simulink library "casper_library_delays"  (Simulink 7.2)
settings: Solver=ode45  SolverMode=SingleTasking  StartTime=0.0  StopTime=10.0  RelTol=1e-3
libraries: xbsIndex_r4 x378, casper_library_misc x18, casper_library_delays x16, xbsReplacements_r4 x5, casper_library_multipliers x4, casper_library_downconverter x2
(part 3 of 5)

== system casper_library_delays/finedelay_fstop_prog_cordic/CORDIC_SINCOS2 ==
  note: The CORDIC algorithm is implemented in 3 steps.
      |
      | Step 1: Coarse Angle Rotation.  The algorithm converges only for angles between -pi/2 and pi/2. If  z > pi/2, the input angle is reflected
      |  to the 1st quadrant by subtracting pi/2 from the input angle. When z < -pi/2, the input angle is reflected back to the 3rd quadrant by adding
      | pi/2 to the input angle .
      |
      | Step 2: Fine Angle Rotation.  By setting x equal to 1/1.646760 and y equal to 0, the rotational mode CORDIC processor yields cosine and sine
      | of the input angle Z.
      |
      | Step 3: Angle Correction. If there was a reflection applied in Step 1, this step applies the appropriate correction .
  z : Inport
  CORDIC Fine Angle PE : Subsystem  mask(CORDIC parallel PE){}
      mask init:
      | [bg,fg] = xlcmap('XBlock',0);
      | iPos = get_param(gcb,'Position');
      | iWidth=iPos(3)-iPos(1); iHeight=iPos(4)-iPos(2);
      | iCx=iWidth/2;
      | iCy=iHeight/2;
      | [logoX, logoY] = xlogo(iPos);
      mask Display:
      | patch([0 iWidth iWidth 0],[0 0 iHeight iHeight] , bg);
      | patch(logoX,logoY , fg);
      | port_label('input',1,'x');
      | port_label('input',2,'y');
      | port_label('input',3,'z');
      | port_label('output',1,'X');
      | port_label('output',2,'Y');
      | plot([0 0 iWidth iWidth 0], [0 iHeight iHeight 0 0]);
  Constant : xbsIndex_r4/Constant  const=1/1.646760  gui_display_data_type=Fixed-point  arith_type=Signed (2's comp)  n_bits=pe_nbits  bin_pt=pe_binpt  preci_type=Single  exp_width=8  frac_width=24  explicit_period=off  period=1  equ=P=C  opselect=C  inp2=PCIN>>17  opr=+  inp1=P  carry=CIN  dbl_ovrd=off  block_type=constant
      settings: block_version=VER_STRING_GOES_HERE
  Constant1 : xbsIndex_r4/Constant  const=0  gui_display_data_type=Fixed-point  arith_type=Signed (2's comp)  n_bits=pe_nbits  bin_pt=pe_binpt  preci_type=Single  exp_width=8  frac_width=24  explicit_period=off  period=1  equ=P=C  opselect=C  inp2=PCIN>>17  opr=+  inp1=P  carry=CIN  dbl_ovrd=off  block_type=constant
      settings: block_version=VER_STRING_GOES_HERE
  Delay1 : xbsIndex_r4/Delay  rst=off  infoeditControl=Selection of Reset will increase slice count due to use of real FFs and instead of SRLs  en=off  latency=sum(pipeline)+2  dbl_ovrd=off  reg_retiming=on  block_type=delay
      settings: infoedit="Delay line having  configurable length.<P><P>Hardware notes: A delay line is a chain, each link of which is an SRL16 followed by a flip-flop. If register retiming is enabled, the delay line is a chain of flip-flops."  xl_area=[1 1 0 1 0 0 0]  block_version=VER_STRING_GOES_HERE
  Delay4 : xbsIndex_r4/Delay  rst=off  infoeditControl=Selection of Reset will increase slice count due to use of real FFs and instead of SRLs  en=off  latency=sum(pipeline)+1  dbl_ovrd=off  reg_retiming=on  block_type=delay
      settings: infoedit="Delay line having  configurable length.<P><P>Hardware notes: A delay line is a chain, each link of which is an SRL16 followed by a flip-flop. If register retiming is enabled, the delay line is a chain of flip-flops."  xl_area=[1 1 0 1 0 0 0]  block_version=VER_STRING_GOES_HERE
  Quadrant Correct : Subsystem
      mask init:
      | [bg,fg] = xlcmap('XBlock',0);
      | iPos = get_param(gcb,'Position');
      | iWidth=iPos(3)-iPos(1); iHeight=iPos(4)-iPos(2);
      | iCx=iWidth/2;
      | iCy=iHeight/2;
      | [logoX, logoY] = xlogo(iPos);
      mask Display:
      | patch([0 iWidth iWidth 0],[0 0 iHeight iHeight] , bg);
      | patch(logoX,logoY , fg);
      | port_label('input',1,'x');
      | port_label('input',2,'y');
      | port_label('input',3,'angle_map');
      | port_label('input',4,'sgn(z)');
      | port_label('output',1,'cos');
      | port_label('output',2,'sin');
      | plot([0 0 iWidth iWidth 0], [0 iHeight iHeight 0 0]);
  Quadrant Map : Subsystem
      mask init:
      | [bg,fg] = xlcmap('XBlock',0);
      | iPos = get_param(gcb,'Position');
      | iWidth=iPos(3)-iPos(1); iHeight=iPos(4)-iPos(2);
      | iCx=iWidth/2;
      | iCy=iHeight/2;
      | [logoX, logoY] = xlogo(iPos);
      mask Display:
      | patch([0 iWidth iWidth 0],[0 0 iHeight iHeight] , bg);
      | patch(logoX,logoY , fg);
      | port_label('input',1,'z');
      | port_label('output',1,'z');
      | port_label('output',2,'angle_map');
      | port_label('output',3,'sgn(z)');
      | plot([0 0 iWidth iWidth 0], [0 iHeight iHeight 0 0]);
  cos : Outport
  sin : Outport  Port=2
  wires:
  CORDIC Fine Angle PE/1(X) -> Quadrant Correct/1(cos)
  CORDIC Fine Angle PE/2(Y) -> Quadrant Correct/2(sin)
  Delay1/1 -> Quadrant Correct/4(sgn(z))
  Delay4/1 -> Quadrant Correct/3(angle_map)
  z/1 -> Quadrant Map/1(z)
  Quadrant Map/2(angle_map) -> Delay4/1
  Quadrant Map/3(sgn_z) -> Delay1/1
  Quadrant Map/1(Z) -> CORDIC Fine Angle PE/3(z)
  Constant/1 -> CORDIC Fine Angle PE/1(x)
  Constant1/1 -> CORDIC Fine Angle PE/2(y)
  Quadrant Correct/2(sine) -> sin/1
  Quadrant Correct/1(cosine) -> cos/1

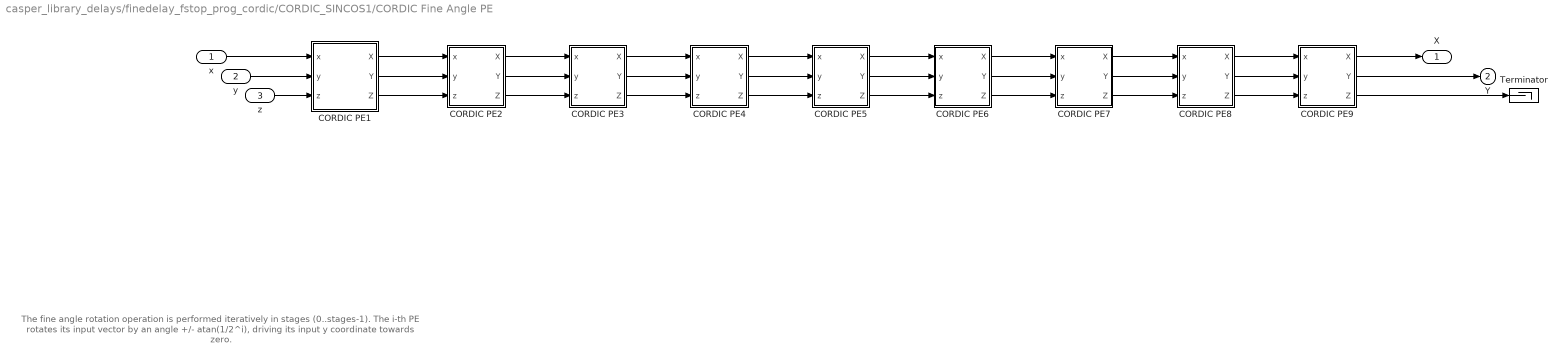
== system casper_library_delays/finedelay_fstop_prog_cordic/CORDIC_SINCOS1/CORDIC Fine Angle PE ==
  note: The fine angle rotation operation is performed iteratively in stages (0..stages-1).
      | The i-th PE rotates its input vector by an angle +/- atan(1/2^i), driving its input y coordinate towards zero.
  x : Inport
  y : Inport  Port=2
  z : Inport  Port=3
  CORDIC PE1 : Subsystem  mask(CORDIC iteration PE){ii=0, pe_nbits=pe_nbits, pe_binpt=pe_binpt, epsilon_k_fcn=atan, epsilon_k=, pipeline=pipeline(1,1)}
      mask prompts: ii "Iteration Index ii"; pe_nbits "Number of X,Y,Z Bits"; pe_binpt "X,Y,Z Binary Point Position"; epsilon_k_fcn "Epsilon_k Function"; pipeline "Pipeline Latency"
      mask init:
      | [bg,fg] = xlcmap('XBlock',0);
      | iPos = get_param(gcb,'Position');
      | iWidth=iPos(3)-iPos(1); iHeight=iPos(4)-iPos(2);
      | iCx=iWidth/2;
      | iCy=iHeight/2;
      | [logoX, logoY] = xlogo(iPos);
      | 
      | set_param(gcb, 'LinkStatus', 'none');
      | switch epsilon_k_fcn
      |   case 1
      |     epsilon_k = atan(1/2^ii);
      |   case 2
      |     epsilon_k = atanh(1/2^ii);
      | end
      mask StyleString: edit,edit,edit,popup(atan|atanh),edit,edit
      mask Display:
      | patch([0 iWidth iWidth 0],[0 0 iHeight iHeight] , bg);
      | patch(logoX,logoY , fg);
      | port_label('input',1,'x');
      | port_label('input',2,'y');
      | port_label('input',3,'z');
      | port_label('output',1,'X');
      | port_label('output',2,'Y');
      | port_label('output',3,'Z');
      | plot([0 0 iWidth iWidth 0], [0 iHeight iHeight 0 0]);
  CORDIC PE2 : Subsystem  mask(CORDIC iteration PE){ii=1, pe_nbits=pe_nbits, pe_binpt=pe_binpt, epsilon_k_fcn=atan, epsilon_k=, pipeline=pipeline(1,2)}
      mask prompts: ii "Iteration Index ii"; pe_nbits "Number of X,Y,Z Bits"; pe_binpt "X,Y,Z Binary Point Position"; epsilon_k_fcn "Epsilon_k Function"; pipeline "Pipeline Latency"
      mask init: same as casper_library_delays/finedelay_fstop_prog_cordic/CORDIC_SINCOS1/CORDIC Fine Angle PE/CORDIC PE1
      mask StyleString: edit,edit,edit,popup(atan|atanh),edit,edit
      mask Display:
      | patch([0 iWidth iWidth 0],[0 0 iHeight iHeight] , bg);
      | patch(logoX,logoY , fg);
      | port_label('input',1,'x');
      | port_label('input',2,'y');
      | port_label('input',3,'z');
      | port_label('output',1,'X');
      | port_label('output',2,'Y');
      | port_label('output',3,'Z');
      | plot([0 0 iWidth iWidth 0], [0 iHeight iHeight 0 0]);
  CORDIC PE3 : Subsystem  mask(CORDIC iteration PE){ii=2, pe_nbits=pe_nbits, pe_binpt=pe_binpt, epsilon_k_fcn=atan, epsilon_k=, pipeline=pipeline(1,3)}
      mask prompts: ii "Iteration Index ii"; pe_nbits "Number of X,Y,Z Bits"; pe_binpt "X,Y,Z Binary Point Position"; epsilon_k_fcn "Epsilon_k Function"; pipeline "Pipeline Latency"
      mask init: same as casper_library_delays/finedelay_fstop_prog_cordic/CORDIC_SINCOS1/CORDIC Fine Angle PE/CORDIC PE1
      mask StyleString: edit,edit,edit,popup(atan|atanh),edit,edit
      mask Display:
      | patch([0 iWidth iWidth 0],[0 0 iHeight iHeight] , bg);
      | patch(logoX,logoY , fg);
      | port_label('input',1,'x');
      | port_label('input',2,'y');
      | port_label('input',3,'z');
      | port_label('output',1,'X');
      | port_label('output',2,'Y');
      | port_label('output',3,'Z');
      | plot([0 0 iWidth iWidth 0], [0 iHeight iHeight 0 0]);
  CORDIC PE4 : Subsystem  mask(CORDIC iteration PE){ii=3, pe_nbits=pe_nbits, pe_binpt=pe_binpt, epsilon_k_fcn=atan, epsilon_k=, pipeline=pipeline(1,4)}
      mask prompts: ii "Iteration Index ii"; pe_nbits "Number of X,Y,Z Bits"; pe_binpt "X,Y,Z Binary Point Position"; epsilon_k_fcn "Epsilon_k Function"; pipeline "Pipeline Latency"
      mask init: same as casper_library_delays/finedelay_fstop_prog_cordic/CORDIC_SINCOS1/CORDIC Fine Angle PE/CORDIC PE1
      mask StyleString: edit,edit,edit,popup(atan|atanh),edit,edit
      mask Display:
      | patch([0 iWidth iWidth 0],[0 0 iHeight iHeight] , bg);
      | patch(logoX,logoY , fg);
      | port_label('input',1,'x');
      | port_label('input',2,'y');
      | port_label('input',3,'z');
      | port_label('output',1,'X');
      | port_label('output',2,'Y');
      | port_label('output',3,'Z');
      | plot([0 0 iWidth iWidth 0], [0 iHeight iHeight 0 0]);
  CORDIC PE5 : Subsystem  mask(CORDIC iteration PE){ii=4, pe_nbits=pe_nbits, pe_binpt=pe_binpt, epsilon_k_fcn=atan, epsilon_k=, pipeline=pipeline(1,5)}
      mask prompts: ii "Iteration Index ii"; pe_nbits "Number of X,Y,Z Bits"; pe_binpt "X,Y,Z Binary Point Position"; epsilon_k_fcn "Epsilon_k Function"; pipeline "Pipeline Latency"
      mask init: same as casper_library_delays/finedelay_fstop_prog_cordic/CORDIC_SINCOS1/CORDIC Fine Angle PE/CORDIC PE1
      mask StyleString: edit,edit,edit,popup(atan|atanh),edit,edit
      mask Display:
      | patch([0 iWidth iWidth 0],[0 0 iHeight iHeight] , bg);
      | patch(logoX,logoY , fg);
      | port_label('input',1,'x');
      | port_label('input',2,'y');
      | port_label('input',3,'z');
      | port_label('output',1,'X');
      | port_label('output',2,'Y');
      | port_label('output',3,'Z');
      | plot([0 0 iWidth iWidth 0], [0 iHeight iHeight 0 0]);
  CORDIC PE6 : Subsystem  mask(CORDIC iteration PE){ii=5, pe_nbits=pe_nbits, pe_binpt=pe_binpt, epsilon_k_fcn=atan, epsilon_k=, pipeline=pipeline(1,6)}
      mask prompts: ii "Iteration Index ii"; pe_nbits "Number of X,Y,Z Bits"; pe_binpt "X,Y,Z Binary Point Position"; epsilon_k_fcn "Epsilon_k Function"; pipeline "Pipeline Latency"
      mask init: same as casper_library_delays/finedelay_fstop_prog_cordic/CORDIC_SINCOS1/CORDIC Fine Angle PE/CORDIC PE1
      mask StyleString: edit,edit,edit,popup(atan|atanh),edit,edit
      mask Display:
      | patch([0 iWidth iWidth 0],[0 0 iHeight iHeight] , bg);
      | patch(logoX,logoY , fg);
      | port_label('input',1,'x');
      | port_label('input',2,'y');
      | port_label('input',3,'z');
      | port_label('output',1,'X');
      | port_label('output',2,'Y');
      | port_label('output',3,'Z');
      | plot([0 0 iWidth iWidth 0], [0 iHeight iHeight 0 0]);
  CORDIC PE7 : Subsystem  mask(CORDIC iteration PE){ii=6, pe_nbits=pe_nbits, pe_binpt=pe_binpt, epsilon_k_fcn=atan, epsilon_k=, pipeline=pipeline(1,7)}
      mask prompts: ii "Iteration Index ii"; pe_nbits "Number of X,Y,Z Bits"; pe_binpt "X,Y,Z Binary Point Position"; epsilon_k_fcn "Epsilon_k Function"; pipeline "Pipeline Latency"
      mask init: same as casper_library_delays/finedelay_fstop_prog_cordic/CORDIC_SINCOS1/CORDIC Fine Angle PE/CORDIC PE1
      mask StyleString: edit,edit,edit,popup(atan|atanh),edit,edit
      mask Display:
      | patch([0 iWidth iWidth 0],[0 0 iHeight iHeight] , bg);
      | patch(logoX,logoY , fg);
      | port_label('input',1,'x');
      | port_label('input',2,'y');
      | port_label('input',3,'z');
      | port_label('output',1,'X');
      | port_label('output',2,'Y');
      | port_label('output',3,'Z');
      | plot([0 0 iWidth iWidth 0], [0 iHeight iHeight 0 0]);
  CORDIC PE8 : Subsystem  mask(CORDIC iteration PE){ii=7, pe_nbits=pe_nbits, pe_binpt=pe_binpt, epsilon_k_fcn=atan, epsilon_k=, pipeline=pipeline(1,8)}
      mask prompts: ii "Iteration Index ii"; pe_nbits "Number of X,Y,Z Bits"; pe_binpt "X,Y,Z Binary Point Position"; epsilon_k_fcn "Epsilon_k Function"; pipeline "Pipeline Latency"
      mask init: same as casper_library_delays/finedelay_fstop_prog_cordic/CORDIC_SINCOS1/CORDIC Fine Angle PE/CORDIC PE1
      mask StyleString: edit,edit,edit,popup(atan|atanh),edit,edit
      mask Display:
      | patch([0 iWidth iWidth 0],[0 0 iHeight iHeight] , bg);
      | patch(logoX,logoY , fg);
      | port_label('input',1,'x');
      | port_label('input',2,'y');
      | port_label('input',3,'z');
      | port_label('output',1,'X');
      | port_label('output',2,'Y');
      | port_label('output',3,'Z');
      | plot([0 0 iWidth iWidth 0], [0 iHeight iHeight 0 0]);
  CORDIC PE9 : Subsystem  mask(CORDIC iteration PE){ii=8, pe_nbits=pe_nbits, pe_binpt=pe_binpt, epsilon_k_fcn=atan, epsilon_k=, pipeline=pipeline(1,9)}
      mask prompts: ii "Iteration Index ii"; pe_nbits "Number of X,Y,Z Bits"; pe_binpt "X,Y,Z Binary Point Position"; epsilon_k_fcn "Epsilon_k Function"; pipeline "Pipeline Latency"
      mask init: same as casper_library_delays/finedelay_fstop_prog_cordic/CORDIC_SINCOS1/CORDIC Fine Angle PE/CORDIC PE1
      mask StyleString: edit,edit,edit,popup(atan|atanh),edit,edit
      mask Display:
      | patch([0 iWidth iWidth 0],[0 0 iHeight iHeight] , bg);
      | patch(logoX,logoY , fg);
      | port_label('input',1,'x');
      | port_label('input',2,'y');
      | port_label('input',3,'z');
      | port_label('output',1,'X');
      | port_label('output',2,'Y');
      | port_label('output',3,'Z');
      | plot([0 0 iWidth iWidth 0], [0 iHeight iHeight 0 0]);
  Terminator : Terminator
  X : Outport
  Y : Outport  Port=2
  wires:
  CORDIC PE1/1(X) -> CORDIC PE2/1(x)
  CORDIC PE1/2(Y) -> CORDIC PE2/2(y)
  CORDIC PE1/3(Z) -> CORDIC PE2/3(z)
  CORDIC PE2/1(X) -> CORDIC PE3/1(x)
  CORDIC PE2/2(Y) -> CORDIC PE3/2(y)
  CORDIC PE2/3(Z) -> CORDIC PE3/3(z)
  CORDIC PE3/1(X) -> CORDIC PE4/1(x)
  CORDIC PE3/2(Y) -> CORDIC PE4/2(y)
  CORDIC PE3/3(Z) -> CORDIC PE4/3(z)
  CORDIC PE4/1(X) -> CORDIC PE5/1(x)
  CORDIC PE4/2(Y) -> CORDIC PE5/2(y)
  CORDIC PE4/3(Z) -> CORDIC PE5/3(z)
  CORDIC PE5/1(X) -> CORDIC PE6/1(x)
  CORDIC PE5/2(Y) -> CORDIC PE6/2(y)
  CORDIC PE5/3(Z) -> CORDIC PE6/3(z)
  CORDIC PE6/1(X) -> CORDIC PE7/1(x)
  CORDIC PE6/2(Y) -> CORDIC PE7/2(y)
  CORDIC PE6/3(Z) -> CORDIC PE7/3(z)
  CORDIC PE7/1(X) -> CORDIC PE8/1(x)
  CORDIC PE7/2(Y) -> CORDIC PE8/2(y)
  CORDIC PE7/3(Z) -> CORDIC PE8/3(z)
  CORDIC PE8/1(X) -> CORDIC PE9/1(x)
  CORDIC PE8/2(Y) -> CORDIC PE9/2(y)
  CORDIC PE8/3(Z) -> CORDIC PE9/3(z)
  x/1 -> CORDIC PE1/1(x)
  y/1 -> CORDIC PE1/2(y)
  z/1 -> CORDIC PE1/3(z)
  CORDIC PE9/1(X) -> X/1
  CORDIC PE9/2(Y) -> Y/1
  CORDIC PE9/3(Z) -> Terminator/1

== system casper_library_delays/finedelay_fstop_prog_cordic/CORDIC_SINCOS1/Quadrant Correct ==
  note: Angle Correction:
      |
      | IF z > pi/2: using z = t + pi/2, then
      |    sin (z ) = sin(t).cos(pi/2) + cos(t).sin(pi/2) = cos(t)
      |    cos (z ) = cos(t).cos(pi/2) - sin(t).sin(pi/2) = -sin(t)
      |
      | IF z < pi/2: using z = t - pi/2, then
      |    sin (z ) = sin(t).cos(-pi/2) + cos(t).sin(-pi/2) = -cos(t)
      |    cos (z ) = cos(t).cos(-pi/2) - sin(t).sin(-pi/2) = sin(t)
  cos : Inport
  sin : Inport  Port=2
  angle_map : Inport  Port=3
  sgn(z) : Inport  Port=4
  Mux : xbsIndex_r4/Mux  inputs=2  en=off  latency=1  precision=User Defined  arith_type="Signed  (2's comp)"  n_bits=pe_nbits  bin_pt=pe_binpt  quantization=Truncate  overflow=Wrap  dbl_ovrd=off  block_type=mux
      settings: xl_area=[8 16 0 16 0 0 0]  block_version=VER_STRING_GOES_HERE
  Mux1 : xbsIndex_r4/Mux  inputs=2  en=off  latency=1  precision=User Defined  arith_type="Signed  (2's comp)"  n_bits=pe_nbits  bin_pt=pe_binpt  quantization=Truncate  overflow=Wrap  dbl_ovrd=off  block_type=mux
      settings: xl_area=[8 16 0 16 0 0 0]  block_version=VER_STRING_GOES_HERE
  Mux2 : xbsIndex_r4/Mux  inputs=2  en=off  latency=0  precision=User Defined  arith_type="Signed  (2's comp)"  n_bits=pe_nbits  bin_pt=pe_binpt  quantization=Truncate  overflow=Wrap  dbl_ovrd=off  block_type=mux
      settings: xl_area=[8 0 0 16 0 0 0]  block_version=VER_STRING_GOES_HERE
  Mux3 : xbsIndex_r4/Mux  inputs=2  en=off  latency=0  precision=User Defined  arith_type="Signed  (2's comp)"  n_bits=pe_nbits  bin_pt=pe_binpt  quantization=Truncate  overflow=Wrap  dbl_ovrd=off  block_type=mux
      settings: xl_area=[8 0 0 16 0 0 0]  block_version=VER_STRING_GOES_HERE
  Negate1 : xbsIndex_r4/Negate  precision=User Defined  arith_type="Signed  (2's comp)"  n_bits=pe_nbits  bin_pt=pe_binpt  quantization=Truncate  overflow=Wrap  en=off  latency=0  dbl_ovrd=off  block_type=negate
      settings: xl_area=[8 0 0 16 0 0 0]  block_version=VER_STRING_GOES_HERE
  Negate2 : xbsIndex_r4/Negate  precision=User Defined  arith_type="Signed  (2's comp)"  n_bits=pe_nbits  bin_pt=pe_binpt  quantization=Truncate  overflow=Wrap  en=off  latency=0  dbl_ovrd=off  block_type=negate
      settings: xl_area=[8 0 0 16 0 0 0]  block_version=VER_STRING_GOES_HERE
  cosine : Outport
  sine : Outport  Port=2
  wires:
  cos/1 -> Mux/2, Negate1/1, Mux2/2
  sin/1 -> Mux1/2, Negate2/1, Mux3/3
  Mux/1 -> cosine/1
  Mux1/1 -> sine/1
  angle_map/1 -> Mux/1, Mux1/1
  Mux3/1 -> Mux/3
  sgn(z)/1 -> Mux2/1, Mux3/1
  Mux2/1 -> Mux1/3
  Negate1/1 -> Mux2/3
  Negate2/1 -> Mux3/2

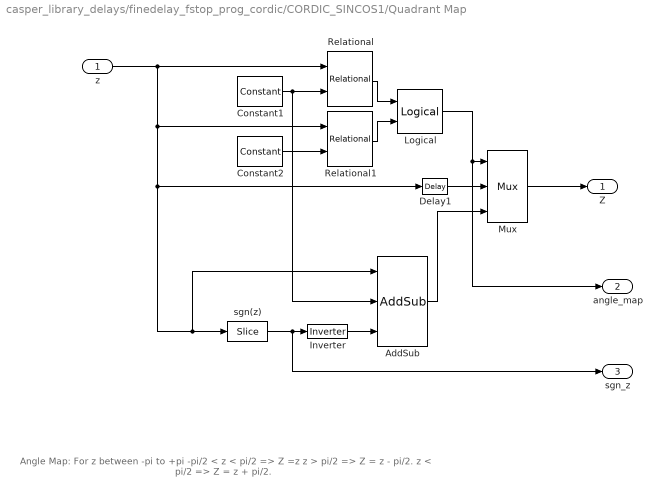
== system casper_library_delays/finedelay_fstop_prog_cordic/CORDIC_SINCOS1/Quadrant Map ==
  note: Angle Map: For z between -pi to +pi
      |
      |  -pi/2 < z  < pi/2  =>  Z =z
      |             z > pi/2   =>  Z = z - pi/2.
      |             z < pi/2   =>  Z = z + pi/2.
  z : Inport
  AddSub : xbsIndex_r4/AddSub  mode=Addition or Subtraction  use_carryin=off  use_carryout=off  en=off  latency=1  precision=User Defined  arith_type="Signed  (2's comp)"  n_bits=pe_nbits  bin_pt=pe_binpt  quantization=Truncate  overflow=Wrap  dbl_ovrd=off  use_behavioral_HDL=on  hw_selection=Fabric  pipelined=off  use_rpm=off  block_type=addsub
      settings: xl_area=[8 16 0 16 0 0 0]  block_version=VER_STRING_GOES_HERE
  Constant1 : xbsIndex_r4/Constant  const=pi/2  gui_display_data_type=Fixed-point  arith_type=Signed (2's comp)  n_bits=pe_nbits  bin_pt=pe_binpt  preci_type=Single  exp_width=8  frac_width=24  explicit_period=off  period=1  equ=P=C  opselect=C  inp2=PCIN>>17  opr=+  inp1=P  carry=CIN  dbl_ovrd=off  block_type=constant
      settings: block_version=VER_STRING_GOES_HERE
  Constant2 : xbsIndex_r4/Constant  const=-pi/2  gui_display_data_type=Fixed-point  arith_type=Signed (2's comp)  n_bits=pe_nbits  bin_pt=pe_binpt  preci_type=Single  exp_width=8  frac_width=24  explicit_period=off  period=1  equ=P=C  opselect=C  inp2=PCIN>>17  opr=+  inp1=P  carry=CIN  dbl_ovrd=off  block_type=constant
      settings: block_version=VER_STRING_GOES_HERE
  Delay1 : xbsIndex_r4/Delay  rst=off  infoeditControl=Selection of Reset will increase slice count due to use of real FFs and instead of SRLs  en=off  latency=1  dbl_ovrd=off  reg_retiming=on  block_type=delay
      settings: infoedit="Delay line having  configurable length.<P><P>Hardware notes: A delay line is a chain, each link of which is an SRL16 followed by a flip-flop. If register retiming is enabled, the delay line is a chain of flip-flops."  xl_area=[8 16 0 0 0 0 0]  block_version=VER_STRING_GOES_HERE
  Inverter : xbsIndex_r4/Inverter  en=off  latency=0  dbl_ovrd=off  block_type=inv
      settings: xl_area=[1 0 0 1 0 0 0]  block_version=VER_STRING_GOES_HERE
  Logical : xbsIndex_r4/Logical  logical_function=OR  inputs=2  en=off  latency=0  precision=Full  arith_type=Unsigned  n_bits=8  bin_pt=2  align_bp=on  dbl_ovrd=off  block_type=logical
      settings: xl_area=[1 0 0 1 0 0 0]  block_version=VER_STRING_GOES_HERE
  Mux : xbsIndex_r4/Mux  inputs=2  en=off  latency=1  precision=User Defined  arith_type="Signed  (2's comp)"  n_bits=pe_nbits  bin_pt=pe_binpt  quantization=Truncate  overflow=Wrap  dbl_ovrd=off  block_type=mux
      settings: xl_area=[8 16 0 16 0 0 0]  block_version=VER_STRING_GOES_HERE
  Relational : xbsIndex_r4/Relational  mode=a>b  en=off  latency=1  dbl_ovrd=off  block_type=relational
      settings: xl_area=[8 1 0 16 0 0 0]  block_version=VER_STRING_GOES_HERE
  Relational1 : xbsIndex_r4/Relational  mode=a<b  en=off  latency=1  dbl_ovrd=off  block_type=relational
      settings: xl_area=[8 1 0 16 0 0 0]  block_version=VER_STRING_GOES_HERE
  sgn(z) : xbsIndex_r4/Slice  nbits=1  boolean_output=on  mode=Upper Bit Location + Width  bit1=0  base1=MSB of Input  bit0=0  base0=LSB of Input  dbl_ovrd=off  block_type=slice
      settings: infoedit="Extracts a given range of bits from each input sample and presents it at the output.  The output type is ordinarily unsigned with binary point at zero, but can be Boolean when the slice is one bit wide.<P><P>Hardware notes: In hardware this block costs nothing."  block_version=VER_STRING_GOES_HERE
  Z : Outport
  angle_map : Outport  Port=2
  sgn_z : Outport  Port=3
  wires:
  z/1 -> Relational1/1, Delay1/1, sgn(z)/1, AddSub/1, Relational/1
  Mux/1 -> Z/1
  sgn(z)/1 -> sgn_z/1, Inverter/1
  Constant1/1 -> Relational/2, AddSub/2
  Constant2/1 -> Relational1/2
  Relational/1 -> Logical/1
  Relational1/1 -> Logical/2
  Logical/1 -> Mux/1, angle_map/1
  Delay1/1 -> Mux/2
  AddSub/1 -> Mux/3
  Inverter/1 -> AddSub/3

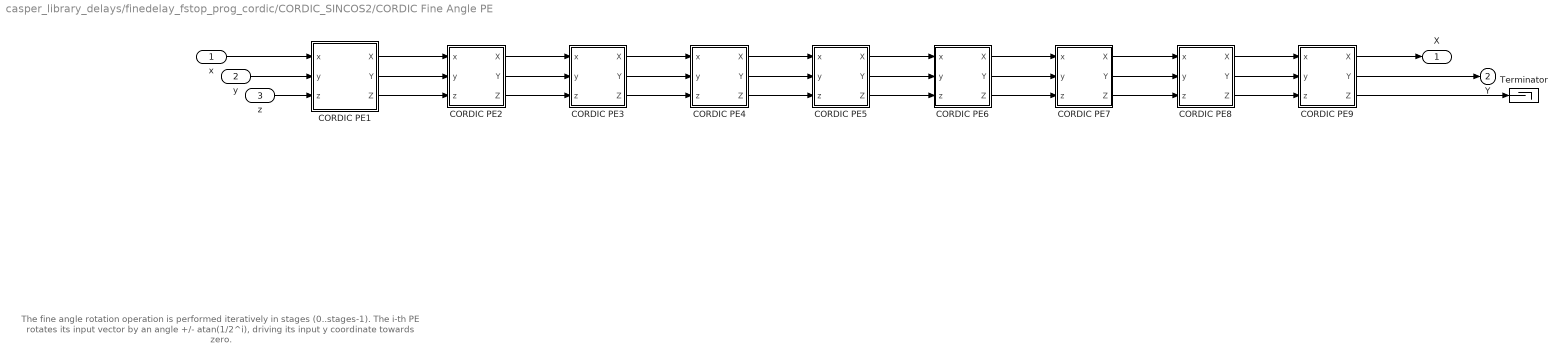
== system casper_library_delays/finedelay_fstop_prog_cordic/CORDIC_SINCOS2/CORDIC Fine Angle PE ==
  note: The fine angle rotation operation is performed iteratively in stages (0..stages-1).
      | The i-th PE rotates its input vector by an angle +/- atan(1/2^i), driving its input y coordinate towards zero.
  x : Inport
  y : Inport  Port=2
  z : Inport  Port=3
  CORDIC PE1 : Subsystem  mask(CORDIC iteration PE){ii=0, pe_nbits=pe_nbits, pe_binpt=pe_binpt, epsilon_k_fcn=atan, epsilon_k=, pipeline=pipeline(1,1)}
      mask prompts: ii "Iteration Index ii"; pe_nbits "Number of X,Y,Z Bits"; pe_binpt "X,Y,Z Binary Point Position"; epsilon_k_fcn "Epsilon_k Function"; pipeline "Pipeline Latency"
      mask init: same as casper_library_delays/finedelay_fstop_prog_cordic/CORDIC_SINCOS1/CORDIC Fine Angle PE/CORDIC PE1
      mask StyleString: edit,edit,edit,popup(atan|atanh),edit,edit
      mask Display:
      | patch([0 iWidth iWidth 0],[0 0 iHeight iHeight] , bg);
      | patch(logoX,logoY , fg);
      | port_label('input',1,'x');
      | port_label('input',2,'y');
      | port_label('input',3,'z');
      | port_label('output',1,'X');
      | port_label('output',2,'Y');
      | port_label('output',3,'Z');
      | plot([0 0 iWidth iWidth 0], [0 iHeight iHeight 0 0]);
  CORDIC PE2 : Subsystem  mask(CORDIC iteration PE){ii=1, pe_nbits=pe_nbits, pe_binpt=pe_binpt, epsilon_k_fcn=atan, epsilon_k=, pipeline=pipeline(1,2)}
      mask prompts: ii "Iteration Index ii"; pe_nbits "Number of X,Y,Z Bits"; pe_binpt "X,Y,Z Binary Point Position"; epsilon_k_fcn "Epsilon_k Function"; pipeline "Pipeline Latency"
      mask init: same as casper_library_delays/finedelay_fstop_prog_cordic/CORDIC_SINCOS1/CORDIC Fine Angle PE/CORDIC PE1
      mask StyleString: edit,edit,edit,popup(atan|atanh),edit,edit
      mask Display:
      | patch([0 iWidth iWidth 0],[0 0 iHeight iHeight] , bg);
      | patch(logoX,logoY , fg);
      | port_label('input',1,'x');
      | port_label('input',2,'y');
      | port_label('input',3,'z');
      | port_label('output',1,'X');
      | port_label('output',2,'Y');
      | port_label('output',3,'Z');
      | plot([0 0 iWidth iWidth 0], [0 iHeight iHeight 0 0]);
  CORDIC PE3 : Subsystem  mask(CORDIC iteration PE){ii=2, pe_nbits=pe_nbits, pe_binpt=pe_binpt, epsilon_k_fcn=atan, epsilon_k=, pipeline=pipeline(1,3)}
      mask prompts: ii "Iteration Index ii"; pe_nbits "Number of X,Y,Z Bits"; pe_binpt "X,Y,Z Binary Point Position"; epsilon_k_fcn "Epsilon_k Function"; pipeline "Pipeline Latency"
      mask init: same as casper_library_delays/finedelay_fstop_prog_cordic/CORDIC_SINCOS1/CORDIC Fine Angle PE/CORDIC PE1
      mask StyleString: edit,edit,edit,popup(atan|atanh),edit,edit
      mask Display:
      | patch([0 iWidth iWidth 0],[0 0 iHeight iHeight] , bg);
      | patch(logoX,logoY , fg);
      | port_label('input',1,'x');
      | port_label('input',2,'y');
      | port_label('input',3,'z');
      | port_label('output',1,'X');
      | port_label('output',2,'Y');
      | port_label('output',3,'Z');
      | plot([0 0 iWidth iWidth 0], [0 iHeight iHeight 0 0]);
  CORDIC PE4 : Subsystem  mask(CORDIC iteration PE){ii=3, pe_nbits=pe_nbits, pe_binpt=pe_binpt, epsilon_k_fcn=atan, epsilon_k=, pipeline=pipeline(1,4)}
      mask prompts: ii "Iteration Index ii"; pe_nbits "Number of X,Y,Z Bits"; pe_binpt "X,Y,Z Binary Point Position"; epsilon_k_fcn "Epsilon_k Function"; pipeline "Pipeline Latency"
      mask init: same as casper_library_delays/finedelay_fstop_prog_cordic/CORDIC_SINCOS1/CORDIC Fine Angle PE/CORDIC PE1
      mask StyleString: edit,edit,edit,popup(atan|atanh),edit,edit
      mask Display:
      | patch([0 iWidth iWidth 0],[0 0 iHeight iHeight] , bg);
      | patch(logoX,logoY , fg);
      | port_label('input',1,'x');
      | port_label('input',2,'y');
      | port_label('input',3,'z');
      | port_label('output',1,'X');
      | port_label('output',2,'Y');
      | port_label('output',3,'Z');
      | plot([0 0 iWidth iWidth 0], [0 iHeight iHeight 0 0]);
  CORDIC PE5 : Subsystem  mask(CORDIC iteration PE){ii=4, pe_nbits=pe_nbits, pe_binpt=pe_binpt, epsilon_k_fcn=atan, epsilon_k=, pipeline=pipeline(1,5)}
      mask prompts: ii "Iteration Index ii"; pe_nbits "Number of X,Y,Z Bits"; pe_binpt "X,Y,Z Binary Point Position"; epsilon_k_fcn "Epsilon_k Function"; pipeline "Pipeline Latency"
      mask init: same as casper_library_delays/finedelay_fstop_prog_cordic/CORDIC_SINCOS1/CORDIC Fine Angle PE/CORDIC PE1
      mask StyleString: edit,edit,edit,popup(atan|atanh),edit,edit
      mask Display:
      | patch([0 iWidth iWidth 0],[0 0 iHeight iHeight] , bg);
      | patch(logoX,logoY , fg);
      | port_label('input',1,'x');
      | port_label('input',2,'y');
      | port_label('input',3,'z');
      | port_label('output',1,'X');
      | port_label('output',2,'Y');
      | port_label('output',3,'Z');
      | plot([0 0 iWidth iWidth 0], [0 iHeight iHeight 0 0]);
  CORDIC PE6 : Subsystem  mask(CORDIC iteration PE){ii=5, pe_nbits=pe_nbits, pe_binpt=pe_binpt, epsilon_k_fcn=atan, epsilon_k=, pipeline=pipeline(1,6)}
      mask prompts: ii "Iteration Index ii"; pe_nbits "Number of X,Y,Z Bits"; pe_binpt "X,Y,Z Binary Point Position"; epsilon_k_fcn "Epsilon_k Function"; pipeline "Pipeline Latency"
      mask init: same as casper_library_delays/finedelay_fstop_prog_cordic/CORDIC_SINCOS1/CORDIC Fine Angle PE/CORDIC PE1
      mask StyleString: edit,edit,edit,popup(atan|atanh),edit,edit
      mask Display:
      | patch([0 iWidth iWidth 0],[0 0 iHeight iHeight] , bg);
      | patch(logoX,logoY , fg);
      | port_label('input',1,'x');
      | port_label('input',2,'y');
      | port_label('input',3,'z');
      | port_label('output',1,'X');
      | port_label('output',2,'Y');
      | port_label('output',3,'Z');
      | plot([0 0 iWidth iWidth 0], [0 iHeight iHeight 0 0]);
  CORDIC PE7 : Subsystem  mask(CORDIC iteration PE){ii=6, pe_nbits=pe_nbits, pe_binpt=pe_binpt, epsilon_k_fcn=atan, epsilon_k=, pipeline=pipeline(1,7)}
      mask prompts: ii "Iteration Index ii"; pe_nbits "Number of X,Y,Z Bits"; pe_binpt "X,Y,Z Binary Point Position"; epsilon_k_fcn "Epsilon_k Function"; pipeline "Pipeline Latency"
      mask init: same as casper_library_delays/finedelay_fstop_prog_cordic/CORDIC_SINCOS1/CORDIC Fine Angle PE/CORDIC PE1
      mask StyleString: edit,edit,edit,popup(atan|atanh),edit,edit
      mask Display:
      | patch([0 iWidth iWidth 0],[0 0 iHeight iHeight] , bg);
      | patch(logoX,logoY , fg);
      | port_label('input',1,'x');
      | port_label('input',2,'y');
      | port_label('input',3,'z');
      | port_label('output',1,'X');
      | port_label('output',2,'Y');
      | port_label('output',3,'Z');
      | plot([0 0 iWidth iWidth 0], [0 iHeight iHeight 0 0]);
  CORDIC PE8 : Subsystem  mask(CORDIC iteration PE){ii=7, pe_nbits=pe_nbits, pe_binpt=pe_binpt, epsilon_k_fcn=atan, epsilon_k=, pipeline=pipeline(1,8)}
      mask prompts: ii "Iteration Index ii"; pe_nbits "Number of X,Y,Z Bits"; pe_binpt "X,Y,Z Binary Point Position"; epsilon_k_fcn "Epsilon_k Function"; pipeline "Pipeline Latency"
      mask init: same as casper_library_delays/finedelay_fstop_prog_cordic/CORDIC_SINCOS1/CORDIC Fine Angle PE/CORDIC PE1
      mask StyleString: edit,edit,edit,popup(atan|atanh),edit,edit
      mask Display:
      | patch([0 iWidth iWidth 0],[0 0 iHeight iHeight] , bg);
      | patch(logoX,logoY , fg);
      | port_label('input',1,'x');
      | port_label('input',2,'y');
      | port_label('input',3,'z');
      | port_label('output',1,'X');
      | port_label('output',2,'Y');
      | port_label('output',3,'Z');
      | plot([0 0 iWidth iWidth 0], [0 iHeight iHeight 0 0]);
  CORDIC PE9 : Subsystem  mask(CORDIC iteration PE){ii=8, pe_nbits=pe_nbits, pe_binpt=pe_binpt, epsilon_k_fcn=atan, epsilon_k=, pipeline=pipeline(1,9)}
      mask prompts: ii "Iteration Index ii"; pe_nbits "Number of X,Y,Z Bits"; pe_binpt "X,Y,Z Binary Point Position"; epsilon_k_fcn "Epsilon_k Function"; pipeline "Pipeline Latency"
      mask init: same as casper_library_delays/finedelay_fstop_prog_cordic/CORDIC_SINCOS1/CORDIC Fine Angle PE/CORDIC PE1
      mask StyleString: edit,edit,edit,popup(atan|atanh),edit,edit
      mask Display:
      | patch([0 iWidth iWidth 0],[0 0 iHeight iHeight] , bg);
      | patch(logoX,logoY , fg);
      | port_label('input',1,'x');
      | port_label('input',2,'y');
      | port_label('input',3,'z');
      | port_label('output',1,'X');
      | port_label('output',2,'Y');
      | port_label('output',3,'Z');
      | plot([0 0 iWidth iWidth 0], [0 iHeight iHeight 0 0]);
  Terminator : Terminator
  X : Outport
  Y : Outport  Port=2
  wires:
  CORDIC PE1/1(X) -> CORDIC PE2/1(x)
  CORDIC PE1/2(Y) -> CORDIC PE2/2(y)
  CORDIC PE1/3(Z) -> CORDIC PE2/3(z)
  CORDIC PE2/1(X) -> CORDIC PE3/1(x)
  CORDIC PE2/2(Y) -> CORDIC PE3/2(y)
  CORDIC PE2/3(Z) -> CORDIC PE3/3(z)
  CORDIC PE3/1(X) -> CORDIC PE4/1(x)
  CORDIC PE3/2(Y) -> CORDIC PE4/2(y)
  CORDIC PE3/3(Z) -> CORDIC PE4/3(z)
  CORDIC PE4/1(X) -> CORDIC PE5/1(x)
  CORDIC PE4/2(Y) -> CORDIC PE5/2(y)
  CORDIC PE4/3(Z) -> CORDIC PE5/3(z)
  CORDIC PE5/1(X) -> CORDIC PE6/1(x)
  CORDIC PE5/2(Y) -> CORDIC PE6/2(y)
  CORDIC PE5/3(Z) -> CORDIC PE6/3(z)
  CORDIC PE6/1(X) -> CORDIC PE7/1(x)
  CORDIC PE6/2(Y) -> CORDIC PE7/2(y)
  CORDIC PE6/3(Z) -> CORDIC PE7/3(z)
  CORDIC PE7/1(X) -> CORDIC PE8/1(x)
  CORDIC PE7/2(Y) -> CORDIC PE8/2(y)
  CORDIC PE7/3(Z) -> CORDIC PE8/3(z)
  CORDIC PE8/1(X) -> CORDIC PE9/1(x)
  CORDIC PE8/2(Y) -> CORDIC PE9/2(y)
  CORDIC PE8/3(Z) -> CORDIC PE9/3(z)
  x/1 -> CORDIC PE1/1(x)
  y/1 -> CORDIC PE1/2(y)
  z/1 -> CORDIC PE1/3(z)
  CORDIC PE9/1(X) -> X/1
  CORDIC PE9/2(Y) -> Y/1
  CORDIC PE9/3(Z) -> Terminator/1

== system casper_library_delays/finedelay_fstop_prog_cordic/CORDIC_SINCOS2/Quadrant Correct ==
  note: Angle Correction:
      |
      | IF z > pi/2: using z = t + pi/2, then
      |    sin (z ) = sin(t).cos(pi/2) + cos(t).sin(pi/2) = cos(t)
      |    cos (z ) = cos(t).cos(pi/2) - sin(t).sin(pi/2) = -sin(t)
      |
      | IF z < pi/2: using z = t - pi/2, then
      |    sin (z ) = sin(t).cos(-pi/2) + cos(t).sin(-pi/2) = -cos(t)
      |    cos (z ) = cos(t).cos(-pi/2) - sin(t).sin(-pi/2) = sin(t)
  cos : Inport
  sin : Inport  Port=2
  angle_map : Inport  Port=3
  sgn(z) : Inport  Port=4
  Mux : xbsIndex_r4/Mux  inputs=2  en=off  latency=1  precision=User Defined  arith_type="Signed  (2's comp)"  n_bits=pe_nbits  bin_pt=pe_binpt  quantization=Truncate  overflow=Wrap  dbl_ovrd=off  block_type=mux
      settings: xl_area=[8 16 0 16 0 0 0]  block_version=VER_STRING_GOES_HERE
  Mux1 : xbsIndex_r4/Mux  inputs=2  en=off  latency=1  precision=User Defined  arith_type="Signed  (2's comp)"  n_bits=pe_nbits  bin_pt=pe_binpt  quantization=Truncate  overflow=Wrap  dbl_ovrd=off  block_type=mux
      settings: xl_area=[8 16 0 16 0 0 0]  block_version=VER_STRING_GOES_HERE
  Mux2 : xbsIndex_r4/Mux  inputs=2  en=off  latency=0  precision=User Defined  arith_type="Signed  (2's comp)"  n_bits=pe_nbits  bin_pt=pe_binpt  quantization=Truncate  overflow=Wrap  dbl_ovrd=off  block_type=mux
      settings: xl_area=[8 0 0 16 0 0 0]  block_version=VER_STRING_GOES_HERE
  Mux3 : xbsIndex_r4/Mux  inputs=2  en=off  latency=0  precision=User Defined  arith_type="Signed  (2's comp)"  n_bits=pe_nbits  bin_pt=pe_binpt  quantization=Truncate  overflow=Wrap  dbl_ovrd=off  block_type=mux
      settings: xl_area=[8 0 0 16 0 0 0]  block_version=VER_STRING_GOES_HERE
  Negate1 : xbsIndex_r4/Negate  precision=User Defined  arith_type="Signed  (2's comp)"  n_bits=pe_nbits  bin_pt=pe_binpt  quantization=Truncate  overflow=Wrap  en=off  latency=0  dbl_ovrd=off  block_type=negate
      settings: xl_area=[8 0 0 16 0 0 0]  block_version=VER_STRING_GOES_HERE
  Negate2 : xbsIndex_r4/Negate  precision=User Defined  arith_type="Signed  (2's comp)"  n_bits=pe_nbits  bin_pt=pe_binpt  quantization=Truncate  overflow=Wrap  en=off  latency=0  dbl_ovrd=off  block_type=negate
      settings: xl_area=[8 0 0 16 0 0 0]  block_version=VER_STRING_GOES_HERE
  cosine : Outport
  sine : Outport  Port=2
  wires:
  cos/1 -> Mux/2, Negate1/1, Mux2/2
  sin/1 -> Mux1/2, Negate2/1, Mux3/3
  Mux/1 -> cosine/1
  Mux1/1 -> sine/1
  angle_map/1 -> Mux/1, Mux1/1
  Mux3/1 -> Mux/3
  sgn(z)/1 -> Mux2/1, Mux3/1
  Mux2/1 -> Mux1/3
  Negate1/1 -> Mux2/3
  Negate2/1 -> Mux3/2

== system casper_library_delays/finedelay_fstop_prog_cordic/CORDIC_SINCOS2/Quadrant Map ==
  note: Angle Map: For z between -pi to +pi
      |
      |  -pi/2 < z  < pi/2  =>  Z =z
      |             z > pi/2   =>  Z = z - pi/2.
      |             z < pi/2   =>  Z = z + pi/2.
  z : Inport
  AddSub : xbsIndex_r4/AddSub  mode=Addition or Subtraction  use_carryin=off  use_carryout=off  en=off  latency=1  precision=User Defined  arith_type="Signed  (2's comp)"  n_bits=pe_nbits  bin_pt=pe_binpt  quantization=Truncate  overflow=Wrap  dbl_ovrd=off  use_behavioral_HDL=on  hw_selection=Fabric  pipelined=off  use_rpm=off  block_type=addsub
      settings: xl_area=[8 16 0 16 0 0 0]  block_version=VER_STRING_GOES_HERE
  Constant1 : xbsIndex_r4/Constant  const=pi/2  gui_display_data_type=Fixed-point  arith_type=Signed (2's comp)  n_bits=pe_nbits  bin_pt=pe_binpt  preci_type=Single  exp_width=8  frac_width=24  explicit_period=off  period=1  equ=P=C  opselect=C  inp2=PCIN>>17  opr=+  inp1=P  carry=CIN  dbl_ovrd=off  block_type=constant
      settings: block_version=VER_STRING_GOES_HERE
  Constant2 : xbsIndex_r4/Constant  const=-pi/2  gui_display_data_type=Fixed-point  arith_type=Signed (2's comp)  n_bits=pe_nbits  bin_pt=pe_binpt  preci_type=Single  exp_width=8  frac_width=24  explicit_period=off  period=1  equ=P=C  opselect=C  inp2=PCIN>>17  opr=+  inp1=P  carry=CIN  dbl_ovrd=off  block_type=constant
      settings: block_version=VER_STRING_GOES_HERE
  Delay1 : xbsIndex_r4/Delay  rst=off  infoeditControl=Selection of Reset will increase slice count due to use of real FFs and instead of SRLs  en=off  latency=1  dbl_ovrd=off  reg_retiming=on  block_type=delay
      settings: infoedit="Delay line having  configurable length.<P><P>Hardware notes: A delay line is a chain, each link of which is an SRL16 followed by a flip-flop. If register retiming is enabled, the delay line is a chain of flip-flops."  xl_area=[8 16 0 0 0 0 0]  block_version=VER_STRING_GOES_HERE
  Inverter : xbsIndex_r4/Inverter  en=off  latency=0  dbl_ovrd=off  block_type=inv
      settings: xl_area=[1 0 0 1 0 0 0]  block_version=VER_STRING_GOES_HERE
  Logical : xbsIndex_r4/Logical  logical_function=OR  inputs=2  en=off  latency=0  precision=Full  arith_type=Unsigned  n_bits=8  bin_pt=2  align_bp=on  dbl_ovrd=off  block_type=logical
      settings: xl_area=[1 0 0 1 0 0 0]  block_version=VER_STRING_GOES_HERE
  Mux : xbsIndex_r4/Mux  inputs=2  en=off  latency=1  precision=User Defined  arith_type="Signed  (2's comp)"  n_bits=pe_nbits  bin_pt=pe_binpt  quantization=Truncate  overflow=Wrap  dbl_ovrd=off  block_type=mux
      settings: xl_area=[8 16 0 16 0 0 0]  block_version=VER_STRING_GOES_HERE
  Relational : xbsIndex_r4/Relational  mode=a>b  en=off  latency=1  dbl_ovrd=off  block_type=relational
      settings: xl_area=[8 1 0 16 0 0 0]  block_version=VER_STRING_GOES_HERE
  Relational1 : xbsIndex_r4/Relational  mode=a<b  en=off  latency=1  dbl_ovrd=off  block_type=relational
      settings: xl_area=[8 1 0 16 0 0 0]  block_version=VER_STRING_GOES_HERE
  sgn(z) : xbsIndex_r4/Slice  nbits=1  boolean_output=on  mode=Upper Bit Location + Width  bit1=0  base1=MSB of Input  bit0=0  base0=LSB of Input  dbl_ovrd=off  block_type=slice
      settings: infoedit="Extracts a given range of bits from each input sample and presents it at the output.  The output type is ordinarily unsigned with binary point at zero, but can be Boolean when the slice is one bit wide.<P><P>Hardware notes: In hardware this block costs nothing."  block_version=VER_STRING_GOES_HERE
  Z : Outport
  angle_map : Outport  Port=2
  sgn_z : Outport  Port=3
  wires:
  z/1 -> Relational1/1, Delay1/1, sgn(z)/1, AddSub/1, Relational/1
  Mux/1 -> Z/1
  sgn(z)/1 -> sgn_z/1, Inverter/1
  Constant1/1 -> Relational/2, AddSub/2
  Constant2/1 -> Relational1/2
  Relational/1 -> Logical/1
  Relational1/1 -> Logical/2
  Logical/1 -> Mux/1, angle_map/1
  Delay1/1 -> Mux/2
  AddSub/1 -> Mux/3
  Inverter/1 -> AddSub/3

== system casper_library_delays/finedelay_fstop_prog_cordic/CORDIC_SINCOS1/CORDIC Fine Angle PE/CORDIC PE1 ==
  note: X = x + y if z < 0, otherwise
      |    = x - y
      | Y = y - x if z < 0, otherwise
      |    = y + x
      | Z = z + atan(1/2^i) if z < 0, otherwise
      |    = z - atan(1/2^i)
  x : Inport
  y : Inport  Port=2
  z : Inport  Port=3
  AddSub : xbsIndex_r4/AddSub  mode=Addition or Subtraction  use_carryin=off  use_carryout=off  en=off  latency=pipeline  precision=User Defined  arith_type="Signed  (2's comp)"  n_bits=pe_nbits  bin_pt=pe_binpt  quantization=Truncate  overflow=Wrap  dbl_ovrd=off  use_behavioral_HDL=on  hw_selection=Fabric  pipelined=off  use_rpm=off  block_type=addsub
      settings: xl_area=[8 16 0 16 0 0 0]  block_version=VER_STRING_GOES_HERE
  AddSub1 : xbsIndex_r4/AddSub  mode=Addition or Subtraction  use_carryin=off  use_carryout=off  en=off  latency=pipeline  precision=User Defined  arith_type="Signed  (2's comp)"  n_bits=pe_nbits  bin_pt=pe_binpt  quantization=Truncate  overflow=Wrap  dbl_ovrd=off  use_behavioral_HDL=on  hw_selection=Fabric  pipelined=off  use_rpm=off  block_type=addsub
      settings: xl_area=[8 16 0 16 0 0 0]  block_version=VER_STRING_GOES_HERE
  AddSub2 : xbsIndex_r4/AddSub  mode=Addition or Subtraction  use_carryin=off  use_carryout=off  en=off  latency=pipeline  precision=User Defined  arith_type="Signed  (2's comp)"  n_bits=pe_nbits  bin_pt=pe_binpt  quantization=Truncate  overflow=Wrap  dbl_ovrd=off  use_behavioral_HDL=on  hw_selection=Fabric  pipelined=off  use_rpm=off  block_type=addsub
      settings: xl_area=[8 16 0 16 0 0 0]  block_version=VER_STRING_GOES_HERE
  Constant : xbsIndex_r4/Constant  const=epsilon_k  gui_display_data_type=Fixed-point  arith_type=Signed (2's comp)  n_bits=pe_nbits  bin_pt=pe_binpt  preci_type=Single  exp_width=8  frac_width=24  explicit_period=off  period=1  equ=P=C  opselect=C  inp2=PCIN>>17  opr=+  inp1=P  carry=CIN  dbl_ovrd=off  block_type=constant
      settings: block_version=VER_STRING_GOES_HERE
  Inverter : xbsIndex_r4/Inverter  en=off  latency=0  dbl_ovrd=off  block_type=inv
      settings: xl_area=[1 0 0 1 0 0 0]  block_version=VER_STRING_GOES_HERE
  Shift : xbsIndex_r4/Shift  shift_dir=Right  shift_bits=ii  en=off  latency=0  precision=User Defined  arith_type="Signed  (2's comp)"  n_bits=pe_nbits  bin_pt=pe_binpt  quantization=Truncate  overflow=Wrap  dbl_ovrd=off  block_type=shift
      settings: xl_area=[0 0 0 0 0 0 0]  block_version=VER_STRING_GOES_HERE
  Shift1 : xbsIndex_r4/Shift  shift_dir=Right  shift_bits=ii  en=off  latency=0  precision=User Defined  arith_type="Signed  (2's comp)"  n_bits=pe_nbits  bin_pt=pe_binpt  quantization=Truncate  overflow=Wrap  dbl_ovrd=off  block_type=shift
      settings: xl_area=[0 0 0 0 0 0 0]  block_version=VER_STRING_GOES_HERE
  Slice : xbsIndex_r4/Slice  nbits=1  boolean_output=on  mode=Upper Bit Location + Width  bit1=0  base1=MSB of Input  bit0=0  base0=LSB of Input  dbl_ovrd=off  block_type=slice
      settings: infoedit="Extracts a given range of bits from each input sample and presents it at the output.  The output type is ordinarily unsigned with binary point at zero, but can be Boolean when the slice is one bit wide.<P><P>Hardware notes: In hardware this block costs nothing."  block_version=VER_STRING_GOES_HERE
  X : Outport
  Y : Outport  Port=2
  Z : Outport  Port=3
  wires:
  x/1 -> AddSub/1, Shift/1
  y/1 -> AddSub1/1, Shift1/1
  AddSub/1 -> X/1
  z/1 -> AddSub2/1, Slice/1
  AddSub1/1 -> Y/1
  AddSub2/1 -> Z/1
  Constant/1 -> AddSub2/2
  Shift/1 -> AddSub1/2
  Shift1/1 -> AddSub/2
  Slice/1 -> Inverter/1, AddSub1/3
  Inverter/1 -> AddSub2/3, AddSub/3

== system casper_library_delays/finedelay_fstop_prog_cordic/CORDIC_SINCOS1/CORDIC Fine Angle PE/CORDIC PE2 ==
  note: X = x + y if z < 0, otherwise
      |    = x - y
      | Y = y - x if z < 0, otherwise
      |    = y + x
      | Z = z + atan(1/2^i) if z < 0, otherwise
      |    = z - atan(1/2^i)
  x : Inport
  y : Inport  Port=2
  z : Inport  Port=3
  AddSub : xbsIndex_r4/AddSub  mode=Addition or Subtraction  use_carryin=off  use_carryout=off  en=off  latency=pipeline  precision=User Defined  arith_type="Signed  (2's comp)"  n_bits=pe_nbits  bin_pt=pe_binpt  quantization=Truncate  overflow=Wrap  dbl_ovrd=off  use_behavioral_HDL=on  hw_selection=Fabric  pipelined=off  use_rpm=off  block_type=addsub
      settings: xl_area=[8 16 0 16 0 0 0]  block_version=VER_STRING_GOES_HERE
  AddSub1 : xbsIndex_r4/AddSub  mode=Addition or Subtraction  use_carryin=off  use_carryout=off  en=off  latency=pipeline  precision=User Defined  arith_type="Signed  (2's comp)"  n_bits=pe_nbits  bin_pt=pe_binpt  quantization=Truncate  overflow=Wrap  dbl_ovrd=off  use_behavioral_HDL=on  hw_selection=Fabric  pipelined=off  use_rpm=off  block_type=addsub
      settings: xl_area=[8 16 0 16 0 0 0]  block_version=VER_STRING_GOES_HERE
  AddSub2 : xbsIndex_r4/AddSub  mode=Addition or Subtraction  use_carryin=off  use_carryout=off  en=off  latency=pipeline  precision=User Defined  arith_type="Signed  (2's comp)"  n_bits=pe_nbits  bin_pt=pe_binpt  quantization=Truncate  overflow=Wrap  dbl_ovrd=off  use_behavioral_HDL=on  hw_selection=Fabric  pipelined=off  use_rpm=off  block_type=addsub
      settings: xl_area=[8 16 0 16 0 0 0]  block_version=VER_STRING_GOES_HERE
  Constant : xbsIndex_r4/Constant  const=epsilon_k  gui_display_data_type=Fixed-point  arith_type=Signed (2's comp)  n_bits=pe_nbits  bin_pt=pe_binpt  preci_type=Single  exp_width=8  frac_width=24  explicit_period=off  period=1  equ=P=C  opselect=C  inp2=PCIN>>17  opr=+  inp1=P  carry=CIN  dbl_ovrd=off  block_type=constant
      settings: block_version=VER_STRING_GOES_HERE
  Inverter : xbsIndex_r4/Inverter  en=off  latency=0  dbl_ovrd=off  block_type=inv
      settings: xl_area=[1 0 0 1 0 0 0]  block_version=VER_STRING_GOES_HERE
  Shift : xbsIndex_r4/Shift  shift_dir=Right  shift_bits=ii  en=off  latency=0  precision=User Defined  arith_type="Signed  (2's comp)"  n_bits=pe_nbits  bin_pt=pe_binpt  quantization=Truncate  overflow=Wrap  dbl_ovrd=off  block_type=shift
      settings: xl_area=[0 0 0 0 0 0 0]  block_version=VER_STRING_GOES_HERE
  Shift1 : xbsIndex_r4/Shift  shift_dir=Right  shift_bits=ii  en=off  latency=0  precision=User Defined  arith_type="Signed  (2's comp)"  n_bits=pe_nbits  bin_pt=pe_binpt  quantization=Truncate  overflow=Wrap  dbl_ovrd=off  block_type=shift
      settings: xl_area=[0 0 0 0 0 0 0]  block_version=VER_STRING_GOES_HERE
  Slice : xbsIndex_r4/Slice  nbits=1  boolean_output=on  mode=Upper Bit Location + Width  bit1=0  base1=MSB of Input  bit0=0  base0=LSB of Input  dbl_ovrd=off  block_type=slice
      settings: infoedit="Extracts a given range of bits from each input sample and presents it at the output.  The output type is ordinarily unsigned with binary point at zero, but can be Boolean when the slice is one bit wide.<P><P>Hardware notes: In hardware this block costs nothing."  block_version=VER_STRING_GOES_HERE
  X : Outport
  Y : Outport  Port=2
  Z : Outport  Port=3
  wires:
  Inverter/1 -> AddSub/3, AddSub2/3
  Slice/1 -> AddSub1/3, Inverter/1
  Shift1/1 -> AddSub/2
  Shift/1 -> AddSub1/2
  Constant/1 -> AddSub2/2
  AddSub2/1 -> Z/1
  AddSub1/1 -> Y/1
  z/1 -> Slice/1, AddSub2/1
  AddSub/1 -> X/1
  y/1 -> Shift1/1, AddSub1/1
  x/1 -> Shift/1, AddSub/1

== system casper_library_delays/finedelay_fstop_prog_cordic/CORDIC_SINCOS1/CORDIC Fine Angle PE/CORDIC PE3 ==
  note: X = x + y if z < 0, otherwise
      |    = x - y
      | Y = y - x if z < 0, otherwise
      |    = y + x
      | Z = z + atan(1/2^i) if z < 0, otherwise
      |    = z - atan(1/2^i)
  x : Inport
  y : Inport  Port=2
  z : Inport  Port=3
  AddSub : xbsIndex_r4/AddSub  mode=Addition or Subtraction  use_carryin=off  use_carryout=off  en=off  latency=pipeline  precision=User Defined  arith_type="Signed  (2's comp)"  n_bits=pe_nbits  bin_pt=pe_binpt  quantization=Truncate  overflow=Wrap  dbl_ovrd=off  use_behavioral_HDL=on  hw_selection=Fabric  pipelined=off  use_rpm=off  block_type=addsub
      settings: xl_area=[8 16 0 16 0 0 0]  block_version=VER_STRING_GOES_HERE
  AddSub1 : xbsIndex_r4/AddSub  mode=Addition or Subtraction  use_carryin=off  use_carryout=off  en=off  latency=pipeline  precision=User Defined  arith_type="Signed  (2's comp)"  n_bits=pe_nbits  bin_pt=pe_binpt  quantization=Truncate  overflow=Wrap  dbl_ovrd=off  use_behavioral_HDL=on  hw_selection=Fabric  pipelined=off  use_rpm=off  block_type=addsub
      settings: xl_area=[8 16 0 16 0 0 0]  block_version=VER_STRING_GOES_HERE
  AddSub2 : xbsIndex_r4/AddSub  mode=Addition or Subtraction  use_carryin=off  use_carryout=off  en=off  latency=pipeline  precision=User Defined  arith_type="Signed  (2's comp)"  n_bits=pe_nbits  bin_pt=pe_binpt  quantization=Truncate  overflow=Wrap  dbl_ovrd=off  use_behavioral_HDL=on  hw_selection=Fabric  pipelined=off  use_rpm=off  block_type=addsub
      settings: xl_area=[8 16 0 16 0 0 0]  block_version=VER_STRING_GOES_HERE
  Constant : xbsIndex_r4/Constant  const=epsilon_k  gui_display_data_type=Fixed-point  arith_type=Signed (2's comp)  n_bits=pe_nbits  bin_pt=pe_binpt  preci_type=Single  exp_width=8  frac_width=24  explicit_period=off  period=1  equ=P=C  opselect=C  inp2=PCIN>>17  opr=+  inp1=P  carry=CIN  dbl_ovrd=off  block_type=constant
      settings: block_version=VER_STRING_GOES_HERE
  Inverter : xbsIndex_r4/Inverter  en=off  latency=0  dbl_ovrd=off  block_type=inv
      settings: xl_area=[1 0 0 1 0 0 0]  block_version=VER_STRING_GOES_HERE
  Shift : xbsIndex_r4/Shift  shift_dir=Right  shift_bits=ii  en=off  latency=0  precision=User Defined  arith_type="Signed  (2's comp)"  n_bits=pe_nbits  bin_pt=pe_binpt  quantization=Truncate  overflow=Wrap  dbl_ovrd=off  block_type=shift
      settings: xl_area=[0 0 0 0 0 0 0]  block_version=VER_STRING_GOES_HERE
  Shift1 : xbsIndex_r4/Shift  shift_dir=Right  shift_bits=ii  en=off  latency=0  precision=User Defined  arith_type="Signed  (2's comp)"  n_bits=pe_nbits  bin_pt=pe_binpt  quantization=Truncate  overflow=Wrap  dbl_ovrd=off  block_type=shift
      settings: xl_area=[0 0 0 0 0 0 0]  block_version=VER_STRING_GOES_HERE
  Slice : xbsIndex_r4/Slice  nbits=1  boolean_output=on  mode=Upper Bit Location + Width  bit1=0  base1=MSB of Input  bit0=0  base0=LSB of Input  dbl_ovrd=off  block_type=slice
      settings: infoedit="Extracts a given range of bits from each input sample and presents it at the output.  The output type is ordinarily unsigned with binary point at zero, but can be Boolean when the slice is one bit wide.<P><P>Hardware notes: In hardware this block costs nothing."  block_version=VER_STRING_GOES_HERE
  X : Outport
  Y : Outport  Port=2
  Z : Outport  Port=3
  wires:
  Inverter/1 -> AddSub/3, AddSub2/3
  Slice/1 -> AddSub1/3, Inverter/1
  Shift1/1 -> AddSub/2
  Shift/1 -> AddSub1/2
  Constant/1 -> AddSub2/2
  AddSub2/1 -> Z/1
  AddSub1/1 -> Y/1
  z/1 -> Slice/1, AddSub2/1
  AddSub/1 -> X/1
  y/1 -> Shift1/1, AddSub1/1
  x/1 -> Shift/1, AddSub/1
